simulink model "Roll_Pitch_Double_PID"  (R2026b)
settings: Solver=FixedStepDiscrete  FixedStep=0.01
undefined symbols (not defined in the file): DiscIntNeverNeededParam
libraries: slpidlib x2

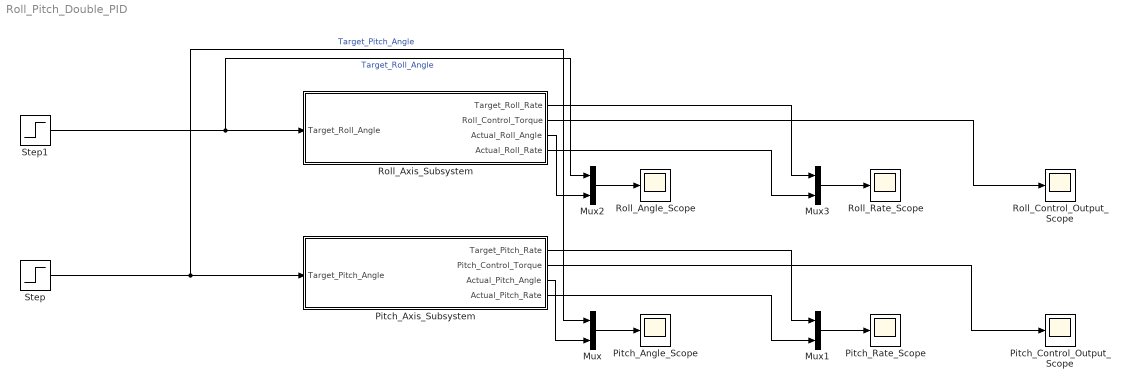
== system Roll_Pitch_Double_PID ==
  Mux{,1..3} (4 alike) : Mux  Inputs=2
  Pitch_Angle_Scope : Scope
      settings: ActiveDisplayYMinimum=-0.058965196206024167  ActiveDisplayYMaximum=0.0065516884673360171
  Pitch_Axis_Subsystem : Subsystem
  Pitch_Control_Output_Scope : Scope
      settings: ActiveDisplayYMinimum=-0.0058906290445815239  ActiveDisplayYMaximum=0.011231109187265192  DataLoggingVariableName=ScopeData2
  Pitch_Rate_Scope : Scope
      settings: ActiveDisplayYMinimum=-0.11782313205433181  ActiveDisplayYMaximum=0.013210637292388569
  Roll_Angle_Scope : Scope
      settings: ActiveDisplayYMinimum=-0.010919480778893362  ActiveDisplayYMaximum=0.09827532701004027  DataLoggingVariableName=ScopeData3
  Roll_Axis_Subsystem : Subsystem
  Roll_Control_Output_Scope : Scope
      settings: ActiveDisplayYMinimum=-0.0010929730690063756  ActiveDisplayYMaximum=0.00981771507430254  DataLoggingVariableName=ScopeData4
  Roll_Rate_Scope : Scope
      settings: ActiveDisplayYMinimum=-0.022017728820647592  ActiveDisplayYMaximum=0.19637188675721967  DataLoggingVariableName=ScopeData5
  Step : Step  FinalValue=-3*pi/180  SampleTime=0.01
  Step1 : Step  FinalValue=5*pi/180  SampleTime=0.01
  wires:
  Step/1 -> Pitch_Axis_Subsystem/1(Target_Pitch_Angle), Mux/1  "Target_Pitch_Angle"
  Mux/1 -> Pitch_Angle_Scope/1
  Mux1/1 -> Pitch_Rate_Scope/1
  Pitch_Axis_Subsystem/1(Target_Pitch_Rate) -> Mux1/1
  Pitch_Axis_Subsystem/2(Pitch_Control_Torque) -> Pitch_Control_Output_Scope/1
  Pitch_Axis_Subsystem/3(Actual_Pitch_Angle) -> Mux/2
  Pitch_Axis_Subsystem/4(Actual_Pitch_Rate) -> Mux1/2
  Roll_Axis_Subsystem/1(Target_Roll_Rate) -> Mux3/1
  Roll_Axis_Subsystem/2(Roll_Control_Torque) -> Roll_Control_Output_Scope/1
  Roll_Axis_Subsystem/3(Actual_Roll_Angle) -> Mux2/2
  Roll_Axis_Subsystem/4(Actual_Roll_Rate) -> Mux3/2
  Mux2/1 -> Roll_Angle_Scope/1
  Mux3/1 -> Roll_Rate_Scope/1
  Step1/1 -> Mux2/1, Roll_Axis_Subsystem/1(Target_Roll_Angle)  "Target_Roll_Angle"

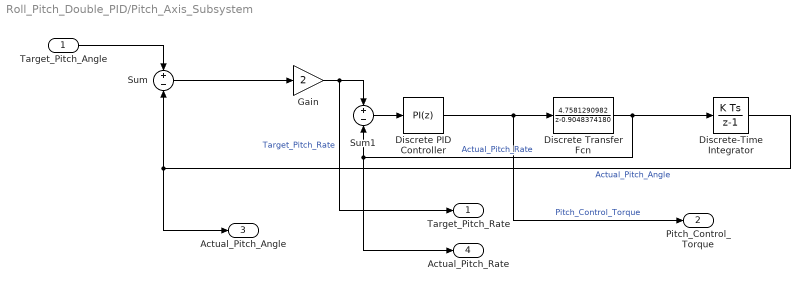
== system Roll_Pitch_Double_PID/Pitch_Axis_Subsystem ==
  Target_Pitch_Angle : Inport
  Discrete Transfer Fcn : DiscreteTransferFcn  Numerator=[0 4.7581290982]  Denominator=[1 -0.9048374180]
  Discrete PID Controller : slpidlib/PID Controller  Controller=PI  Form=Parallel  TimeDomain=Discrete-time  UseExternalTs=off  SampleTime=0.01  IntegratorMethod=Forward Euler  FilterMethod=Forward Euler  ControllerParametersSource=internal  P=0.05  I=0.2  UseKiTs=off  D=0  UseExternalDerivativeSource=off  N=100  UseFilter=on  TunerSelectOption=Transfer Function Based (PID Tuner App)  InitialConditionSource=internal  InitialConditionForIntegrator=0  InitialConditionForFilter=0  DifferentiatorICPrevScaledInput=0  ExternalReset=none  TrackingMode=off  Kt=1  LimitOutput=off  SatLimitsSource=internal  UpperSaturationLimit=inf  LowerSaturationLimit=-inf  LinearizeAsGain=off  AntiWindupMode=none  Kb=1  LimitIntegrator=off  UpperIntegratorSaturationLimit=inf  LowerIntegratorSaturationLimit=-inf  POutMin=[]  POutMax=[]  IOutMin=[]  IOutMax=[]  DOutMin=[]  DOutMax=[]  NOutMin=[]  NOutMax=[]  SumOutMin=[]  SumOutMax=[]  SaturationOutMin=[]  SaturationOutMax=[]  PParamMin=[]  PParamMax=[]  IParamMin=[]  IParamMax=[]  DParamMin=[]  DParamMax=[]  NParamMin=[]  NParamMax=[]  KbParamMin=[]  KbParamMax=[]  KtParamMin=[]  KtParamMax=[]  KbOutMin=[]  KbOutMax=[]  KtOutMin=[]  KtOutMax=[]  IntegratorOutMin=[]  IntegratorOutMax=[]  FilterOutMin=[]  FilterOutMax=[]  SumI1OutMin=[]  SumI1OutMax=[]  SumI2OutMin=[]  SumI2OutMax=[]  SumI3OutMin=[]  SumI3OutMax=[]  SumI4OutMin=[]  SumI4OutMax=[]  SumDOutMin=[]  SumDOutMax=[]  DifferentiatorOutMin=[]  DifferentiatorOutMax=[]  FilterDiffOutCoefMin=[]  FilterDiffOutCoefMax=[]  ReciprocalOutMin=[]  ReciprocalOutMax=[]  SumDenOutMin=[]  SumDenOutMax=[]  SumNumOutMin=[]  SumNumOutMax=[]  DivideOutMin=[]  DivideOutMax=[]  UdiffTsProdOutMin=[]  UdiffTsProdOutMax=[]  NTsProdOutMin=[]  NTsProdOutMax=[]  UintegralTsProdOutMin=[]  UintegralTsProdOutMax=[]  UngainTsProdOutMin=[]  UngainTsProdOutMax=[]  ClampingZeroOutDataTypeStr=Inherit: Inherit via back propagation  ClampingZeroOutMin=[]  ClampingZeroOutMax=[]  FilterDenConstantOutDataTypeStr=Inherit: Inherit via back propagation  FilterDenConstantOutMin=[]  FilterDenConstantOutMax=[]  PCopyOutDataTypeStr=Inherit: Inherit via back propagation  PCopyOutMin=[]  PCopyOutMax=[]  NCopyOutDataTypeStr=Inherit: Inherit via back propagation  NCopyOutMin=[]  NCopyOutMax=[]  IntegratorContinuousStateAttributes=''  IntegratorStateMustResolveToSignalObject=off  IntegratorRTWStateStorageClass=Auto  FilterContinuousStateAttributes=''  FilterStateMustResolveToSignalObject=off  FilterRTWStateStorageClass=Auto  ParallelPVariant=InternalParameters  IdealPVariant=Disabled  IVariant=InternalParameters  DVariant=Disabled  IntegratorVariant=Discrete  SatVariant=Disabled  AWVariant=Passthrough  PCopyVariant=Disabled  TRVariant=Disabled  FdbkBlocksVariant=Forward  IdealPFdbkVariant=Disabled  SatFdbkVariant=Disabled  DerivativeFilterVariant=Disabled  NVariant=Disabled  NCopyVariant=Disabled_SignalSpec  FilterICVariant=Disabled  IntegratorICVariant=InternalICs  ExternalResetVariant=Disabled  TRSumVariant=Passthrough  SumFdbkVariant=Disabled  SumVariant=Sum_PI  TsampFilterVariant=InternalTs  TsampNgainVariant=Passthrough  TsampIntegralVariant=Disabled_SignalSpec  ExternalSaturationOutDataTypeStr=Inherit: Same as second input  DerivativeSourceVariant=Disabled  PreIntVariant=InternalPreInt
      settings: LibrarySourceBlock=simulink/Discrete/Discrete PID Controller
  Discrete-Time Integrator : DiscreteIntegrator  SampleTime=0.01  ICPrevOutput=DiscIntNeverNeededParam  ICPrevScaledInput=DiscIntNeverNeededParam
  Gain : Gain  Gain=2
  Sum : Sum  Inputs=+-
  Sum1 : Sum  Inputs=+-
  Target_Pitch_Rate : Outport
  Pitch_Control_Torque : Outport  Port=2
  Actual_Pitch_Angle : Outport  Port=3
  Actual_Pitch_Rate : Outport  Port=4
  wires:
  Discrete PID Controller/1 -> Pitch_Control_Torque/1, Discrete Transfer Fcn/1  "Pitch_Control_Torque"
  Sum/1 -> Gain/1
  Sum1/1 -> Discrete PID Controller/1
  Target_Pitch_Angle/1 -> Sum/1
  Gain/1 -> Target_Pitch_Rate/1, Sum1/1  "Target_Pitch_Rate"
  Discrete Transfer Fcn/1 -> Actual_Pitch_Rate/1, Sum1/2, Discrete-Time Integrator/1  "Actual_Pitch_Rate"
  Discrete-Time Integrator/1 -> Actual_Pitch_Angle/1, Sum/2  "Actual_Pitch_Angle"

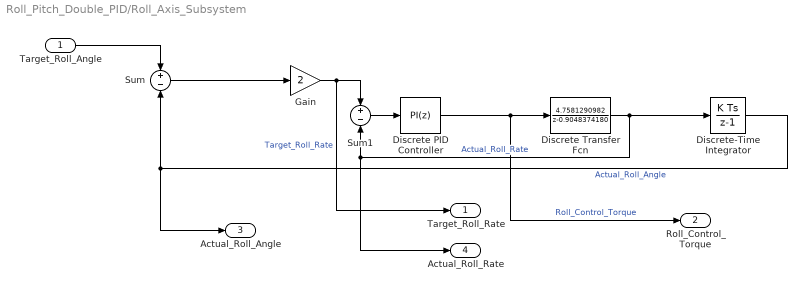
== system Roll_Pitch_Double_PID/Roll_Axis_Subsystem ==
  Target_Roll_Angle : Inport
  Discrete Transfer Fcn : DiscreteTransferFcn  Numerator=[0 4.7581290982]  Denominator=[1 -0.9048374180]
  Discrete PID Controller : slpidlib/PID Controller  Controller=PI  Form=Parallel  TimeDomain=Discrete-time  UseExternalTs=off  SampleTime=0.01  IntegratorMethod=Forward Euler  FilterMethod=Forward Euler  ControllerParametersSource=internal  P=0.05  I=0.2  UseKiTs=off  D=0  UseExternalDerivativeSource=off  N=100  UseFilter=on  TunerSelectOption=Transfer Function Based (PID Tuner App)  InitialConditionSource=internal  InitialConditionForIntegrator=0  InitialConditionForFilter=0  DifferentiatorICPrevScaledInput=0  ExternalReset=none  TrackingMode=off  Kt=1  LimitOutput=off  SatLimitsSource=internal  UpperSaturationLimit=inf  LowerSaturationLimit=-inf  LinearizeAsGain=off  AntiWindupMode=none  Kb=1  LimitIntegrator=off  UpperIntegratorSaturationLimit=inf  LowerIntegratorSaturationLimit=-inf  POutMin=[]  POutMax=[]  IOutMin=[]  IOutMax=[]  DOutMin=[]  DOutMax=[]  NOutMin=[]  NOutMax=[]  SumOutMin=[]  SumOutMax=[]  SaturationOutMin=[]  SaturationOutMax=[]  PParamMin=[]  PParamMax=[]  IParamMin=[]  IParamMax=[]  DParamMin=[]  DParamMax=[]  NParamMin=[]  NParamMax=[]  KbParamMin=[]  KbParamMax=[]  KtParamMin=[]  KtParamMax=[]  KbOutMin=[]  KbOutMax=[]  KtOutMin=[]  KtOutMax=[]  IntegratorOutMin=[]  IntegratorOutMax=[]  FilterOutMin=[]  FilterOutMax=[]  SumI1OutMin=[]  SumI1OutMax=[]  SumI2OutMin=[]  SumI2OutMax=[]  SumI3OutMin=[]  SumI3OutMax=[]  SumI4OutMin=[]  SumI4OutMax=[]  SumDOutMin=[]  SumDOutMax=[]  DifferentiatorOutMin=[]  DifferentiatorOutMax=[]  FilterDiffOutCoefMin=[]  FilterDiffOutCoefMax=[]  ReciprocalOutMin=[]  ReciprocalOutMax=[]  SumDenOutMin=[]  SumDenOutMax=[]  SumNumOutMin=[]  SumNumOutMax=[]  DivideOutMin=[]  DivideOutMax=[]  UdiffTsProdOutMin=[]  UdiffTsProdOutMax=[]  NTsProdOutMin=[]  NTsProdOutMax=[]  UintegralTsProdOutMin=[]  UintegralTsProdOutMax=[]  UngainTsProdOutMin=[]  UngainTsProdOutMax=[]  ClampingZeroOutDataTypeStr=Inherit: Inherit via back propagation  ClampingZeroOutMin=[]  ClampingZeroOutMax=[]  FilterDenConstantOutDataTypeStr=Inherit: Inherit via back propagation  FilterDenConstantOutMin=[]  FilterDenConstantOutMax=[]  PCopyOutDataTypeStr=Inherit: Inherit via back propagation  PCopyOutMin=[]  PCopyOutMax=[]  NCopyOutDataTypeStr=Inherit: Inherit via back propagation  NCopyOutMin=[]  NCopyOutMax=[]  IntegratorContinuousStateAttributes=''  IntegratorStateMustResolveToSignalObject=off  IntegratorRTWStateStorageClass=Auto  FilterContinuousStateAttributes=''  FilterStateMustResolveToSignalObject=off  FilterRTWStateStorageClass=Auto  ParallelPVariant=InternalParameters  IdealPVariant=Disabled  IVariant=InternalParameters  DVariant=Disabled  IntegratorVariant=Discrete  SatVariant=Disabled  AWVariant=Passthrough  PCopyVariant=Disabled  TRVariant=Disabled  FdbkBlocksVariant=Forward  IdealPFdbkVariant=Disabled  SatFdbkVariant=Disabled  DerivativeFilterVariant=Disabled  NVariant=Disabled  NCopyVariant=Disabled_SignalSpec  FilterICVariant=Disabled  IntegratorICVariant=InternalICs  ExternalResetVariant=Disabled  TRSumVariant=Passthrough  SumFdbkVariant=Disabled  SumVariant=Sum_PI  TsampFilterVariant=InternalTs  TsampNgainVariant=Passthrough  TsampIntegralVariant=Disabled_SignalSpec  ExternalSaturationOutDataTypeStr=Inherit: Same as second input  DerivativeSourceVariant=Disabled  PreIntVariant=InternalPreInt
      settings: LibrarySourceBlock=simulink/Discrete/Discrete PID Controller
  Discrete-Time Integrator : DiscreteIntegrator  SampleTime=0.01  ICPrevOutput=DiscIntNeverNeededParam  ICPrevScaledInput=DiscIntNeverNeededParam
  Gain : Gain  Gain=2
  Sum : Sum  Inputs=+-
  Sum1 : Sum  Inputs=+-
  Target_Roll_Rate : Outport
  Roll_Control_Torque : Outport  Port=2
  Actual_Roll_Angle : Outport  Port=3
  Actual_Roll_Rate : Outport  Port=4
  wires:
  Discrete PID Controller/1 -> Roll_Control_Torque/1, Discrete Transfer Fcn/1  "Roll_Control_Torque"
  Sum/1 -> Gain/1
  Sum1/1 -> Discrete PID Controller/1
  Target_Roll_Angle/1 -> Sum/1
  Gain/1 -> Target_Roll_Rate/1, Sum1/1  "Target_Roll_Rate"
  Discrete Transfer Fcn/1 -> Actual_Roll_Rate/1, Sum1/2, Discrete-Time Integrator/1  "Actual_Roll_Rate"
  Discrete-Time Integrator/1 -> Actual_Roll_Angle/1, Sum/2  "Actual_Roll_Angle"
